simulink model "test"  (Simulink 7.0)
settings: Solver=FixedStepDiscrete  StartTime=0.0  StopTime=inf  FixedStep=.1  RelTol=1e-3
libraries: dsPICConfigLib x4, dsPICRunTimeLib x1
settings Model: Creator=sicard  LastModifiedBy=atoubi
settings OptimizationCC: InlineParams=on  InlineInvariantSignals=on  EnforceIntegerDowncast=off  StateBitsets=on  DataBitsets=on  UseTempVars=on  ZeroExternalMemoryAtStartup=off  ZeroInternalMemoryAtStartup=off  InitFltsAndDblsToZero=off  OptimizeModelRefInitCode=on  LifeSpan=1
settings DebuggingCC: InheritedTsInSrcMsg=none
settings HardwareCC: ProdBitPerInt=16  ProdIntDivRoundTo=Zero  ProdEndianess=LittleEndian  ProdWordSize=16  ProdHWDeviceType=Microchip->dsPIC33F  TargetHWDeviceType=32-bit Generic  ProdEqTarget=off
settings RTWCC: SystemTargetFile=dsPIC_stf.tlc  GenCodeOnly=on  GenerateMakefile=off  TemplateMakefile=dsPIC_gcc.tmf  PostCodeGenCommand=MplabGetBuildinfo(buildInfo)  Description=Embedded Target for Microchip dsPIC33fxx (real-time)  ProcessScript=dsPIC_stf_make_rtw_hook
settings CodeAppCC: IgnoreCustomStorageClasses=off
settings STFCustomTargetCC: GenFloatMathFcnCalls=ANSI_C  ModelReferenceCompliant=off  IncludeMdlTerminateFcn=off  CombineOutputUpdateFcns=on  ERTCustomFileBanners=on  SupportContinuousTime=off  SupportNonInlinedSFcns=off  SystemTargetFile=dsPIC_stf.tlc
settings ERTTargetCC: GenFloatMathFcnCalls=ANSI_C  ModelReferenceCompliant=off  CompOptLevelCompliant=off  IncludeMdlTerminateFcn=off  ModelStepFunctionPrototypeControlCompliant=off  InlinedParameterPlacement=NonHierarchical  ERTSrcFileBannerTemplate=dsPIC_code_template.cgt  ERTHdrFileBannerTemplate=dsPIC_code_template.cgt  ERTDataSrcFileTemplate=dsPIC_code_template.cgt  ERTDataHdrFileTemplate=dsPIC_code_template.cgt  ERTCustomFileTemplate=dsPIC_main.tlc
settings CustomProperty: DataType=string  Value=33FJ32MC302

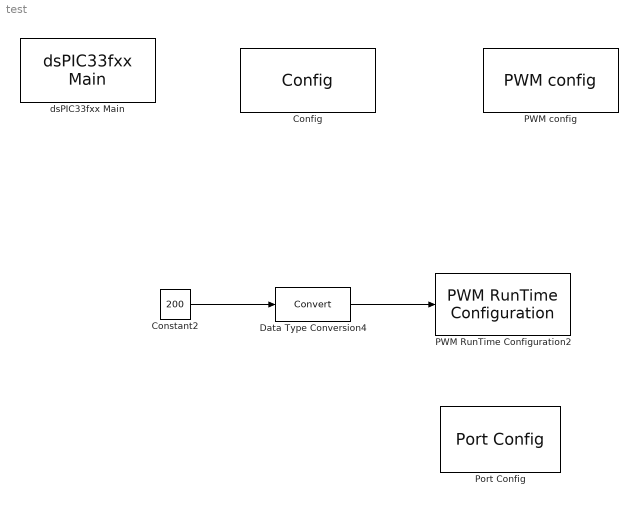
== system test ==
  Config : dsPICConfigLib/Config
  Constant2 : Constant  Value=200  OutDataType=sfix(16)  OutScaling=2^0
  Data Type Conversion4 : DataTypeConversion  OutMin=0  OutMax=65535  OutDataTypeMode=uint16  OutDataType=sfix(16)  OutScaling=2^0
  PWM RunTime Configuration2 : dsPICRunTimeLib/PWM RunTime Configuration  PDCCHOICE=PDC1  OVDCONREQ=off
  PWM config : dsPICConfigLib/PWM config  Priority=-19  PWMSEL=1  PTPER=368  PDC1=368  PDC2=368  PDC3=4  PDC4=58821  PMOD1=complementary output mode  PMOD2=complementary output mode  PMOD3=complementary output mode  PMOD4=complementary output mode  PEN4H=off  PEN3H=on  PEN2H=on  PEN1H=on  PEN4L=off  PEN3L=on  PEN2L=on  PEN1L=on  IUE=off  OSYNC=Output overrides via the PxOVDCON(1) register occur on the next TCY boundary  UDIS=off  PWMINTEN=off  PWMINTP=4  SEVTDIR=Trigger when PWM time base is counting up  SEVTCMP=0  PTEN=on  PTSIDL=off  PTOPS=1  PTCKPS=input clock period is TCY (1:1 prescale)  PTMOD=Free Running mode  PTFREQ=10000  PDC1P=100  PDC2P=100  PDC3P=1  PDC4P=15984  PWMPIN=Control pin state at reset by the module  HPOL=Ative Low  LPOL=Ative Low  DTBPS=Clock period for Dead Time Unit B is TCY  DTB=0  DTAPS=Clock period for Dead Time Unit A is TCY  DTA=0  DTS4A=Dead time provided from Unit A  DTS4I=Dead time provided from Unit A  DTS3A=Dead time provided from Unit A  DTS3I=Dead time provided from Unit A  DTS2A=Dead time provided from Unit A  DTS2I=Dead time provided from Unit A  DTS1A=Dead time provided from Unit A  DTS1I=Dead time provided from Unit A  FAOV4H=Drive PWM output pin Inactive on an external fault input event  FAOV3H=Drive PWM output pin Inactive on an external fault input event  FAOV2H=Drive PWM output pin Inactive on an external fault input event  FAOV1H=Drive PWM output pin Inactive on an external fault input event  FAOV4L=Drive PWM output pin Inactive on an external fault input event  FAOV3L=Drive PWM output pin Inactive on an external fault input event  FAOV2L=Drive PWM output pin Inactive on an external fault input event  FAOV1L=Drive PWM output pin Inactive on an external fault input event  FLTAM=Fault A input pin latches all control pins to the programmed states in PxFLTACON<15:8>  FAEN4=off  FAEN3=off  FAEN2=off  FAEN1=off  FBOV4H=Drive PWM output pin Inactive on an external fault input event  FBOV3H=Drive PWM output pin Inactive on an external fault input event  FBOV2H=Drive PWM output pin Inactive on an external fault input event  FBOV1H=Drive PWM output pin Inactive on an external fault input event  FBOV4L=Drive PWM output pin Inactive on an external fault input event  FBOV3L=Drive PWM output pin Inactive on an external fault input event  FBOV2L=Drive PWM output pin Inactive on an external fault input event  FBOV1L=Drive PWM output pin Inactive on an external fault input event  FLTBM=Fault B input pin latches all control pins to the programmed states in PxFLTACON<15:8>  FBEN4=off  FBEN3=off  FBEN2=off  FBEN1=off  POVD4H=off  POUT4H=Drive PWM4H Inactive when POVD4H bit is cleared  POVD4L=off  POUT4L=Drive PWM4L Inactive when POVD4L bit is cleared  POVD3H=off  POUT3H=Drive PWM3H Active when POVD3H bit is cleared  POVD3L=off  POUT3L=Drive PWM3L Active when POVD3L bit is cleared  POVD2H=off  POUT2H=Drive PWM2H Active when POVD2H bit is cleared  POVD2L=off  POUT2L=Drive PWM2L Active when POVD2L bit is cleared  POVD1H=off  POUT1H=Drive PWM1H Active when POVD1H bit is cleared  POVD1L=off  POUT1L=Drive PWM1L Active when POVD1L bit is cleared
  Port Config : dsPICConfigLib/Port Config  portPolarity=Output  selectPort=B  singlePin=on  selectPin=[10 11 12 13 14 15]
  dsPIC33fxx Main : dsPICConfigLib/dsPIC33fxx Main  Priority=-50  PICTYPE=33FJ32MC302  timer=Timer1  OscSrcSel=Primary oscillator (XT HS EC) w/ PLL  Fin=8e6  Fcy=20000000  ReqLpTm=1  PR1=20000  IESO=Enabled  Temperature=Disabled  ClockSwi=Both enabled  Osc2=Digital I/O  OscSel=External clock  FICD=Use PGC1/EMUC1 and PGD1/EMUD1  Wdt=Disabled  WinWdt=Disabled  WdtPre=1:32  WdtPost=1:1  HSCP=code protect off  CodeProtect=Disabled  WriteProtect=Disabled  PLLDIV=38  PLLPRE=0  PLLPOST=1  TMR1PRESCL=0
  wires:
  Data Type Conversion4/1 -> PWM RunTime Configuration2/1
  Constant2/1 -> Data Type Conversion4/1
